simulink model "ASM_Traffic_MultiCore"  (R2026a)
settings: Solver=ode1  StartTime=SIM.tstart.v  StopTime=SIM.tend.v  FixedStep=SIM.StepSize.v
PostLoadFcn:
  | if any(exist('dsrtsu_mdlpostloadfcn', 'file') ~= 0), dsrtsu_mdlpostloadfcn('Execute', bdroot); end
  | try, asm_mdl_postloadfcn(bdroot, 'UpdateModel', 3600); catch, disp(lasterr); end,
InitFcn:
  | , if any(exist('rtifpga_mdlclblib', 'file') ~= 0), rtifpga_mdlclblib('Init', bdroot); end,
  | , if any(exist('dsmpb_private', 'file') ~= 0), dsmpb_private('dsmpb_mdlclblib', 'Init', bdroot); end,
model workspace (MAT data in the model file):
  asmReferencePath = [0 0.01 0.02 0.03 0.04 0.05 0.06 0.07 0.08 0.09 0.1 0.11 ... (350007 elements, 50001x7)]
  roadBounds : Simulink.Parameter (value not decoded)
  safetyAxes : Simulink.Parameter (value not decoded)
undefined symbols (not defined in the file): _to_, a0b2, ASM_BrakeHydraulics_DemoSystems, ASM_VehicleDynamics_DemoSystems, b98103fe8ad365046cd0, BrakeCircuit, controllerConfig, CPT, Crankshaft, DiscIntNeverNeededParam, dsmsi, FinalDriveAssembly, MDL, ModeSignals, mu, Pos_BrakePedal_Maneuver, rad, RefSignals, roadFamilyData, roadFamilyId, s_to_rpm, SIM, SoftECU, Suspension, Tire, Transmission
libraries: ASM_Traffic_lib x135, simulink x98, ASM_Utils_lib x77, ASM_VehicleDynamics_lib x70, ASM_Environment_lib x22, dsmpblib x20, dsmsilib x15, MDLD_Utils_lib x10, ASM_BrakeHydraulics_lib x3, sl_discontinuities x2
(part 4 of 65)

== system ASM_Traffic_MultiCore/ElectricalSystem/SignalInterface ==
  In : Inport
  ASMSignalInterface : Subsystem  mask(ASM_SIGNAL_INTERFACE){LabelTextfield=ElectricalSystem}
      mask prompts: LabelTextfield "Label"
      mask help:
      | The ASMSignalInterface block processes the ASMSignalBus and provides a vector-based interface for each signal (e.g. ModelDesk Plotting).
      |
      | Always push the update button after you have changed the signal bus structure in order to synchronize the signal interface. The update may take a few seconds.
      | A modified model must be reloaded in ModelDesk to keep consistency of ModelDesk and simulation model plot signals. Therefore select ''Update Model'' from the ''Simulation Model'' context menu of the ModelDesk Project Navigator.
      settings: AttributesFormatString=Label: %<LabelTextfield>
      settings: CopyFcn=|
      | try
      |  set_param(gcb,'LinkStatus', 'none')
      | catch
      | end
      mask Help: eval(['asm_modelhelp(gcbh,''tool'',''ASM_Utils_lib'', ''ASMSIGNALINTERFACE'')'])
      mask DialogControl Hint Prompt: For changes of Label first apply change and then push "Update".
      mask DialogControl UpdateButton Prompt: Update
      mask DialogControl UpdateButton Callback: asm_mdld_plot_block_update(bdroot(gcb), 'update', 'current');
      mask DialogControl UpdateAllButton Prompt: Update All
      mask DialogControl UpdateAllButton Callback: asm_mdld_plot_block_update(bdroot(gcb), 'update', 'all');
  Bus Selector Disable Signals : BusSelector  OutputSignals=ExternalModel.Sw_ModelDeskPlottingInterface[0Disabled|1Enabled]
  wires:
  Bus Selector Disable Signals/1 -> ASMSignalInterface/Enable  "<Sw_ModelDeskPlottingInterface[0Disabled|1Enabled]>"
  In/1 -> Bus Selector Disable Signals/1
  [ASMBUS_ElectricalSystem_Plant] -> ASMSignalInterface/1(ASMSignalBus)

== system ASM_Traffic_MultiCore/Engine/Control ==
  note: Engine Basic Control
  Interface_In : Inport
  Plant : Inport  Port=2
  SoftECU_Engine : Subsystem
  UserInterface : Subsystem
  Control : Outport  VectorParamsAs1DForOutWhenUnconnected=off
  wires:
  SoftECU_Engine/1(ASMSignalBus) -> UserInterface/1(In)
  UserInterface/1(Out) -> SoftECU_Engine/1(UserInterface)
  Plant/1 -> SoftECU_Engine/3(Plant)
  SoftECU_Engine/2(Out) -> Control/1
  Interface_In/1 -> SoftECU_Engine/2(Interface_In)

== system ASM_Traffic_MultiCore/Engine/Interface_In ==
  note: Engine Basic
  In : Inport
  Bus Creator : BusCreator  Inputs=1
  Bus Selector2 : BusSelector  OutputSignals=Environment.Plant.Sw_ModelPortBlocks[0Disabled|1Enabled],Environment.Plant.Sw_ModelDeskPlottingInterface[0Disabled|1Enabled],DomainControl.TorqueManager.Control.Ignition_ICE[0Off|1On],DomainControl.TorqueManager.Control.StarterReq_ICE[0Off|1On],Drivetrain.Control.Factor_Trq_Engine_Red[%],VehicleDynamics.Control.Enable_TrqDecrease_Fast_ESP[0|1],VehicleDynamics.Control.Trq_DecreaseRequest_Fast_ESP[Nm],VehicleDynamics.Control.Enable_TrqIncrease_ESP[0|1],VehicleDynamics.Control.Trq_IncreaseRequest_ESP[Nm],VehicleDynamics.Control.Enable_TrqDecrease_Slow_ESP[0|1],VehicleDynamics.Control.Trq_DecreaseRequest_Slow_ESP[Nm],DomainControl.TorqueManager.Control.Trq_Request_ICE[Nm],Driver.Plant.Pos_AccPedal[%],Environment.Plant.Reset_States[0|1],Drivetrain.Plant.n_Engine[rpm],Environment.Plant.State_StartButton[-1PowerOff|0Acc|1PowerOn|2StarterOn],DomainControl.TorqueManager.Control.Vehicle_Topology[-2|-1|0|2],VehicleDynamics.Plant.v_x_Vehicle_CoG[km|h],Drivetrain.Plant.Sw_CrankShaft_Reset[0Disabled|1Enabled],Environment.Plant.Mode_StartButtonState[1Stim|2SoftECU],DomainControl.DriverAssistance.Control.Enable_Trq_Increase_ACC[0|1],DomainControl.DriverAssistance.Control.Trq_IncreaseRequest_ACC[Nm]
  Enable_n_Engine_Idle_Request[0|1] : Constant  Value=0
  ModelSignals : Subsystem
  n_Engine_Idle_Request[rpm] : Constant  Value=0
  Out : Outport  VectorParamsAs1DForOutWhenUnconnected=off
  wires:
  Bus Selector2/2 -> ModelSignals/2(Sw_ModelDeskPlottingInterface[0Disabled|1Enabled])  "<Sw_ModelDeskPlottingInterface[0Disabled|1Enabled]>"
  Bus Selector2/1 -> ModelSignals/1(Sw_ModelPortBlocks[0Disabled|1Enabled])  "<Sw_ModelPortBlocks[0Disabled|1Enabled]>"
  In/1 -> Bus Selector2/1
  Bus Selector2/12 -> ModelSignals/12(Trq_Request_ICE[Nm])  "<Trq_Request_ICE[Nm]>"
  Bus Selector2/22 -> ModelSignals/22(Trq_Request_Extern2[Nm])  "<Trq_IncreaseRequest_ACC[Nm]>"
  Bus Selector2/21 -> ModelSignals/21(Enable_Trq_Request_Extern2[0|1])  "<Enable_Trq_Increase_ACC[0|1]>"
  Bus Selector2/7 -> ModelSignals/7(Trq_Decrease_Request_Fast_ESP[Nm])  "<Trq_DecreaseRequest_Fast_ESP[Nm]>"
  Bus Selector2/6 -> ModelSignals/6(Enable_Trq_Decrease_Fast_ESP[0|1])  "<Enable_TrqDecrease_Fast_ESP[0|1]>"
  Bus Selector2/5 -> ModelSignals/5(Factor_Trq_Engine_Red[%])  "<Factor_Trq_Engine_Red[%]>"
  Bus Selector2/4 -> ModelSignals/4(Sw_StarterReq[0Off|1On])  "<StarterReq_ICE[0Off|1On]>"
  Bus Selector2/3 -> ModelSignals/3(Sw_Ignition[0Off|1On])  "<Ignition_ICE[0Off|1On]>"
  Bus Selector2/11 -> ModelSignals/11(Trq_Request_Extern1[Nm])  "<Trq_DecreaseRequest_Slow_ESP[Nm]>"
  Bus Selector2/10 -> ModelSignals/10(Enable_Trq_Request_Extern1[0|1])  "<Enable_TrqDecrease_Slow_ESP[0|1]>"
  Bus Selector2/9 -> ModelSignals/9(Trq_Increase_Request_Fast_ESP[Nm])  "<Trq_IncreaseRequest_ESP[Nm]>"
  Bus Selector2/8 -> ModelSignals/8(Enable_Trq_Increase_Fast_ESP[0|1])  "<Enable_TrqIncrease_ESP[0|1]>"
  Bus Creator/1 -> Out/1
  Enable_n_Engine_Idle_Request[0|1]/1 -> ModelSignals/23(Enable_n_Engine_Idle_Request[0|1])
  n_Engine_Idle_Request[rpm]/1 -> ModelSignals/24(n_Engine_Idle_Request[rpm])
  Bus Selector2/13 -> ModelSignals/13(Pos_AccPedal_Driver[%])  "<Pos_AccPedal[%]>"
  Bus Selector2/14 -> ModelSignals/14(Reset_States[0|1])  "<Reset_States[0|1]>"
  Bus Selector2/15 -> ModelSignals/15(n_Engine[rpm])  "<n_Engine[rpm]>"
  Bus Selector2/16 -> ModelSignals/16(State_StartButton[-1|0|1|2])  "<State_StartButton[-1PowerOff|0Acc|1PowerOn|2StarterOn]>"
  Bus Selector2/17 -> ModelSignals/17(Vehicle_Topology[-2|-1|0|2])  "<Vehicle_Topology[-2|-1|0|2]>"
  Bus Selector2/18 -> ModelSignals/18(v_x_Vehicle[km|h])  "<v_x_Vehicle_CoG[km|h]>"
  Bus Selector2/19 -> ModelSignals/19(Sw_CrankShaft_Reset[0Disabled|1Enabled])  "<Sw_CrankShaft_Reset[0Disabled|1Enabled]>"
  Bus Selector2/20 -> ModelSignals/20(Mode_StartButtonState[1Stim|2SoftECU])  "<Mode_StartButtonState[1Stim|2SoftECU]>"
  ModelSignals/1(Out) -> Bus Creator/1

== system ASM_Traffic_MultiCore/Engine/Interface_Out ==
  note: Engine Basic
  In : Inport
  Bus Creator2 : BusCreator  Inputs=2
  Bus Selector2 : BusSelector  OutputSignals=Plant.Engine.Trq_Eff_Engine[Nm],Plant.Engine.Trq_Fric_Engine[Nm]
  Bus Selector6 : BusSelector  OutputSignals=Control.State_Engine[0|1|2|3|4],Control.n_Engine_Idle_Set[rpm],Control.Sw_Starter[0Off|1On],Control.Enable_Trq_Shift_Request[0|1],Control.Trq_Shift_Request[Nm]
  Control_ModelSignals : Subsystem
  CrankAngle_Cyl[aTDC] : Constant  Value=0
  EngOP_Num[] : Constant  Value=0
  Plant_ModelSignals : Subsystem
  Pos_AccPedal_Meas[%] : Constant  Value=0
  State_StartStop[1Off|2NotReady|3Ready|4EngStopped] : Constant
  Sw_Replace_Env[0|1] : Constant  Value=0
  T_Ambient[degC] : Constant  Value=23
  T_Coolant_ICE[degC] : Constant  Value=85
  Trq_MeanEff_Engine_Meas[Nm] : Constant  Value=0
  Type_Engine[0Unkown|1Other|2Otto|3Diesel|4Electric] : Constant
  n_Engine_Meas[rpm] : Constant  Value=0
  p_Ambient[Pa] : Constant  Value=1e5
  Out : Outport  VectorParamsAs1DForOutWhenUnconnected=off
  wires:
  CrankAngle_Cyl[aTDC]/1 -> Control_ModelSignals/7(CrankAngle_Cyl[aTDC])
  T_Ambient[degC]/1 -> Control_ModelSignals/9(T_Ambient[degC])
  p_Ambient[Pa]/1 -> Control_ModelSignals/8(p_Ambient[Pa])
  Trq_MeanEff_Engine_Meas[Nm]/1 -> Control_ModelSignals/14(Trq_MeanEff_Engine_Meas[Nm])
  n_Engine_Meas[rpm]/1 -> Control_ModelSignals/13(n_Engine_Meas[rpm])
  Pos_AccPedal_Meas[%]/1 -> Control_ModelSignals/12(Pos_AccPedal_Meas[%])
  EngOP_Num[]/1 -> Control_ModelSignals/11(EngOP_Num[])
  Sw_Replace_Env[0|1]/1 -> Control_ModelSignals/10(Sw_Replace_Env[0|1])
  Bus Selector6/2 -> Control_ModelSignals/2(n_Engine_Idle_Set[rpm])  "<n_Engine_Idle_Set[rpm]>"
  Bus Selector6/1 -> Control_ModelSignals/1(State_ICEngine[0|1|2|3|4])  "<State_Engine[0|1|2|3|4]>"
  State_StartStop[1Off|2NotReady|3Ready|4EngStopped]/1 -> Control_ModelSignals/6(State_StartStop[1Off|2NotReady|3Ready|4EngStopped])
  T_Coolant_ICE[degC]/1 -> Plant_ModelSignals/3(T_Coolant_ICE[degC])
  Bus Selector2/2 -> Plant_ModelSignals/2(Trq_Fric_Engine[Nm])  "<Trq_Fric_Engine[Nm]>"
  In/1 -> Bus Selector6/1, Bus Selector2/1
  Bus Selector2/1 -> Plant_ModelSignals/1(Trq_MeanEff_Engine[Nm])  "<Trq_Eff_Engine[Nm]>"
  Bus Creator2/1 -> Out/1  "Engine"
  Bus Selector6/3 -> Control_ModelSignals/3(Sw_Starter[0Off|1On])  "<Sw_Starter[0Off|1On]>"
  Bus Selector6/4 -> Control_ModelSignals/4(Enable_Trq_Shift_Request[0|1])  "<Enable_Trq_Shift_Request[0|1]>"
  Bus Selector6/5 -> Control_ModelSignals/5(Trq_Shift_Request[Nm])  "<Trq_Shift_Request[Nm]>"
  Control_ModelSignals/1(Out) -> Bus Creator2/1
  Plant_ModelSignals/1(Out) -> Bus Creator2/2
  Type_Engine[0Unkown|1Other|2Otto|3Diesel|4Electric]/1 -> Plant_ModelSignals/4(Type_Engine[0Unkown|1Other|2Otto|3Diesel|4Electric])

== system ASM_Traffic_MultiCore/Engine/Plant ==
  note: Engine Basic
  Interface_In : Inport
  Control : Inport  Port=2
  EngineBasic : Subsystem
  UserInterface : Subsystem
  Plant : Outport  VectorParamsAs1DForOutWhenUnconnected=off
  wires:
  Control/1 -> EngineBasic/3(Control)
  UserInterface/1(Out) -> EngineBasic/1(UserInterface)
  Interface_In/1 -> UserInterface/2(Interface_In), EngineBasic/2(Interface_In)
  EngineBasic/1(ASMSignalBus) -> Plant/1, UserInterface/1(In)

== system ASM_Traffic_MultiCore/Engine/SignalInterface ==
  In : Inport
  ASMSignalInterface : Subsystem  mask(ASM_SIGNAL_INTERFACE){LabelTextfield=Engine}
      mask prompts: LabelTextfield "Label"
      mask help:
      | The ASMSignalInterface block processes the ASMSignalBus and provides a vector-based interface for each signal (e.g. ModelDesk Plotting).
      |
      | Always push the update button after you have changed the signal bus structure in order to synchronize the signal interface. The update may take a few seconds.
      | A modified model must be reloaded in ModelDesk to keep consistency of ModelDesk and simulation model plot signals. Therefore select ''Update Model'' from the ''Simulation Model'' context menu of the ModelDesk Project Navigator.
      settings: AttributesFormatString=Label: %<LabelTextfield>
      settings: CopyFcn=|
      | try
      |  set_param(gcb,'LinkStatus', 'none')
      | catch
      | end
      mask Help: eval(['asm_modelhelp(gcbh,''tool'',''ASM_Utils_lib'', ''ASMSIGNALINTERFACE'')'])
      mask DialogControl Hint Prompt: For changes of Label first apply change and then push "Update".
      mask DialogControl UpdateButton Prompt: Update
      mask DialogControl UpdateButton Callback: asm_mdld_plot_block_update(bdroot(gcb), 'update', 'current');
      mask DialogControl UpdateAllButton Prompt: Update All
      mask DialogControl UpdateAllButton Callback: asm_mdld_plot_block_update(bdroot(gcb), 'update', 'all');
  Bus Creator : BusCreator  Inputs=2
  Bus Selector Disable Signals : BusSelector  OutputSignals=ExternalModel.Sw_ModelPortBlocks[0Disabled|1Enabled],ExternalModel.Sw_ModelDeskPlottingInterface[0Disabled|1Enabled]
  ExternalOutports : Subsystem  TreatAsAtomicUnit=on
  wires:
  Bus Selector Disable Signals/2 -> ASMSignalInterface/Enable  "<Sw_ModelDeskPlottingInterface[0Disabled|1Enabled]>"
  Bus Selector Disable Signals/1 -> ExternalOutports/Enable  "<Sw_ModelPortBlocks[0Disabled|1Enabled]>"
  In/1 -> Bus Selector Disable Signals/1
  Bus Creator/1 -> ASMSignalInterface/1(ASMSignalBus), ExternalOutports/1(In1)
  [ASMBUS_Engine_Control] -> Bus Creator/1
  [ASMBUS_Engine_Plant] -> Bus Creator/2

== system ASM_Traffic_MultiCore/Environment/GroundTruth ==
  note: GroundTruth
  In : Inport
  Bus Creator2 : BusCreator  Inputs=1
  PlantModel : Subsystem
  UserInterface : Subsystem
  Out : Outport  VectorParamsAs1DForOutWhenUnconnected=off
  wires:
  UserInterface/1(Out) -> PlantModel/1(UserInterface)
  In/1 -> PlantModel/2(In), UserInterface/1(Interface_In)
  PlantModel/1(ASMSignalBus) -> UserInterface/2(In), Bus Creator2/1
  Bus Creator2/1 -> Out/1  "GroundTruth"

== system ASM_Traffic_MultiCore/Environment/Interface_In ==
  note: Environment Traffic
  In : Inport
  Bus Creator1 : BusCreator  Inputs=1
  Bus Selector1 : BusSelector  OutputSignals=Environment.Plant.Sw_ModelPortBlocks[0Disabled|1Enabled],Environment.Plant.Sw_ModelDeskPlottingInterface[0Disabled|1Enabled],VehicleDynamics.Plant.Angle_SteeringWheel[deg],VehicleDynamics.Plant.Angle_SteeringWheel_dt[deg|s],VehicleDynamics.Plant.Trq_SteeringWheel[Nm],VehicleDynamics.Plant.r_Dyn_Tire[FL;FR;RL;RR][m],VehicleDynamics.Plant.Coef_RollingRes[FL;FR;RL;RR][],VehicleDynamics.Plant.CorneringStiffness[FL;FR;RL;RR][N],VehicleDynamics.Plant.Pos_Vehicle_CoorSys_E[x;y;z][m],VehicleDynamics.Plant.Angle_Vehicle_CoorSys_E[x;y;z][deg],VehicleDynamics.Plant.s_Vehicle[m],VehicleDynamics.Plant.v_x_Vehicle_CoG[km|h],VehicleDynamics.Plant.v_y_Vehicle_CoG[km|h],VehicleDynamics.Plant.RollRate_Vehicle_CoG[deg|s],VehicleDynamics.Plant.YawRate_Vehicle_CoG[deg|s],VehicleDynamics.Plant.a_y_Vehicle_CoG[m|s2],VehicleDynamics.Plant.RotationMatrix_V_to_E[1x9],VehicleDynamics.Plant.Const_r_unloaded_Tire_Mean[m],VehicleDynamics.Plant.Coef_RollingRes_Mean[],DomainControl.DriverAssistance.Control.AEB[0|1],DomainControl.DriverAssistance.Control.FCW[0|1],Driver.Plant.Pos_AccPedal[%],Driver.Plant.Pos_BrakePedal[%],Driver.Plant.Pos_ClutchPedal[%],Drivetrain.Plant.Gear[],Driver.Plant.SelectorLever[-3T|-2P|-1R|0N|1D],Driver.Plant.s_Preview[m],Driver.Plant.Angle_SteeringWheel[deg],Driver.Plant.t_Preview_vRef_Driver[s],Drivetrain.Plant.Type_Engine_1[0Unkown|1Other|2Otto|3Diesel|4Electric],Drivetrain.Plant.Trq_Engine_1[Nm],Drivetrain.Plant.n_Engine_1[rpm],Drivetrain.Plant.Type_Engine_2[0Unkown|1Other|2Otto|3Diesel|4Electric],Drivetrain.Plant.Trq_Engine_2[Nm],Drivetrain.Plant.n_Engine_2[rpm],VehicleDynamics.Plant.m_TotalVehicle[kg],DomainControl.StartSystem.Control.State_StartButton[-2|-1|0|1|2|3],DomainControl.DriverAssistance.Control.ACC_State[1OFF|2Standby|3ON],DomainControl.DriverAssistance.Control.Driver_Override_ACC_Active[0Off|1On],DomainControl.DriverAssistance.Control.Driver_Override_ACC_Reason[0NoOverride|1BrakePedal|2AccPedal],VehicleDynamics.Plant.omega_Wheel[rad|s],VehicleDynamics.Plant.Slip_x_Wheel[],VehicleDynamics.Plant.Pos_CP_FL_CoorSys_E[x;y][m],VehicleDynamics.Plant.Pos_CP_FR_CoorSys_E[x;y][m],VehicleDynamics.Plant.Pos_CP_RL_CoorSys_E[x;y][m],VehicleDynamics.Plant.Pos_CP_RL2_CoorSys_E[x;y][m],VehicleDynamics.Plant.Pos_CP_RR_CoorSys_E[x;y][m],VehicleDynamics.Plant.Pos_CP_RR2_CoorSys_E[x;y][m],VehicleDynamics.Plant.Pos_CP_R2L_CoorSys_E[x;y][m],VehicleDynamics.Plant.Pos_CP_R2L2_CoorSys_E[x;y][m],VehicleDynamics.Plant.Pos_CP_R2R_CoorSys_E[x;y][m],VehicleDynamics.Plant.Pos_CP_R2R2_CoorSys_E[x;y][m],Drivetrain.Plant.Mode_Transmission[1Manual|2Automatic],Drivetrain.Plant.Mode_Drivetrain[1|2|3|4|5],VehicleDynamics.Plant.Sw_MasterBrakeCylinder_Mode[1linear|2physical|3Booster],VehicleDynamics.Plant.Active_CP_VehDyn[],VehicleDynamics.Plant.Pos_CP_Front_CoorSys_E[x;y][m],VehicleDynamics.Plant.Pos_CP_Rear_CoorSys_E[x;y][m]
  ModelSignals : Subsystem
  Pos_CP_FL2_Trailer_CoorSys_E[x;y][m] : Constant  Value=[0;0]
  Pos_CP_FL_Trailer_CoorSys_E[x;y][m] : Constant  Value=[0;0]
  Pos_CP_FR2_Trailer_CoorSys_E[x;y][m] : Constant  Value=[0;0]
  Pos_CP_FR_Trailer_CoorSys_E[x;y][m] : Constant  Value=[0;0]
  Pos_CP_R2L2_Trailer_CoorSys_E[x;y][m] : Constant  Value=[0;0]
  Pos_CP_R2L_Trailer_CoorSys_E[x;y][m] : Constant  Value=[0;0]
  Pos_CP_R2R2_Trailer_CoorSys_E[x;y][m] : Constant  Value=[0;0]
  Pos_CP_R2R_Trailer_CoorSys_E[x;y][m] : Constant  Value=[0;0]
  Pos_CP_RL2_Trailer_CoorSys_E[x;y][m] : Constant  Value=[0;0]
  Pos_CP_RL_Trailer_CoorSys_E[x;y][m] : Constant  Value=[0;0]
  Pos_CP_RR2_Trailer_CoorSys_E[x;y][m] : Constant  Value=[0;0]
  Pos_CP_RR_Trailer_CoorSys_E[x;y][m] : Constant  Value=[0;0]
  Out : Outport  VectorParamsAs1DForOutWhenUnconnected=off
  wires:
  Bus Creator1/1 -> Out/1  "Interface_In"
  ModelSignals/1(Out) -> Bus Creator1/1
  Pos_CP_FL_Trailer_CoorSys_E[x;y][m]/1 -> ModelSignals/57(Pos_CP_FL_Trailer_CoorSys_E[x;y][m])
  Pos_CP_FL2_Trailer_CoorSys_E[x;y][m]/1 -> ModelSignals/58(Pos_CP_FL2_Trailer_CoorSys_E[x;y][m])
  Pos_CP_FR_Trailer_CoorSys_E[x;y][m]/1 -> ModelSignals/59(Pos_CP_FR_Trailer_CoorSys_E[x;y][m])
  Pos_CP_FR2_Trailer_CoorSys_E[x;y][m]/1 -> ModelSignals/60(Pos_CP_FR2_Trailer_CoorSys_E[x;y][m])
  Pos_CP_RL_Trailer_CoorSys_E[x;y][m]/1 -> ModelSignals/61(Pos_CP_RL_Trailer_CoorSys_E[x;y][m])
  Pos_CP_RL2_Trailer_CoorSys_E[x;y][m]/1 -> ModelSignals/62(Pos_CP_RL2_Trailer_CoorSys_E[x;y][m])
  Pos_CP_RR_Trailer_CoorSys_E[x;y][m]/1 -> ModelSignals/63(Pos_CP_RR_Trailer_CoorSys_E[x;y][m])
  Pos_CP_RR2_Trailer_CoorSys_E[x;y][m]/1 -> ModelSignals/64(Pos_CP_RR2_Trailer_CoorSys_E[x;y][m])
  Pos_CP_R2L_Trailer_CoorSys_E[x;y][m]/1 -> ModelSignals/65(Pos_CP_R2L_Trailer_CoorSys_E[x;y][m])
  Pos_CP_R2L2_Trailer_CoorSys_E[x;y][m]/1 -> ModelSignals/66(Pos_CP_R2L2_Trailer_CoorSys_E[x;y][m])
  Pos_CP_R2R_Trailer_CoorSys_E[x;y][m]/1 -> ModelSignals/67(Pos_CP_R2R_Trailer_CoorSys_E[x;y][m])
  Pos_CP_R2R2_Trailer_CoorSys_E[x;y][m]/1 -> ModelSignals/68(Pos_CP_R2R2_Trailer_CoorSys_E[x;y][m])
  Bus Selector1/1 -> ModelSignals/1(Sw_ModelPortBlocks[0Disabled|1Enabled])  "<Sw_ModelPortBlocks[0Disabled|1Enabled]>"
  Bus Selector1/2 -> ModelSignals/2(Sw_ModelDeskPlottingInterface[0Disabled|1Enabled])  "<Sw_ModelDeskPlottingInterface[0Disabled|1Enabled]>"
  Bus Selector1/3 -> ModelSignals/3(Angle_SteeringWheel_SteeringSystem[deg])  "<Angle_SteeringWheel[deg]>"
  Bus Selector1/4 -> ModelSignals/4(Angle_SteeringWheel_dt_SteeringSystem[deg|s])  "<Angle_SteeringWheel_dt[deg|s]>"
  Bus Selector1/5 -> ModelSignals/5(Trq_SteeringWheel_SteeringSystem[Nm])  "<Trq_SteeringWheel[Nm]>"
  Bus Selector1/6 -> ModelSignals/6(r_Dyn_Tire[FL;FR;RL;RR][m])  "<r_Dyn_Tire[FL;FR;RL;RR][m]>"
  Bus Selector1/7 -> ModelSignals/7(Coef_RollingRes[FL;FR;RL;RR][])  "<Coef_RollingRes[FL;FR;RL;RR][]>"
  Bus Selector1/8 -> ModelSignals/8(CorneringStiffness[FL;FR;RL;RR][N])  "<CorneringStiffness[FL;FR;RL;RR][N]>"
  Bus Selector1/9 -> ModelSignals/9(Pos_Vehicle_CoorSys_E[x;y;z][m])  "<Pos_Vehicle_CoorSys_E[x;y;z][m]>"
  Bus Selector1/10 -> ModelSignals/10(Angle_Vehicle_CoorSys_E[x;y;z][deg])  "<Angle_Vehicle_CoorSys_E[x;y;z][deg]>"
  Bus Selector1/11 -> ModelSignals/11(s_Vehicle[m])  "<s_Vehicle[m]>"
  Bus Selector1/12 -> ModelSignals/12(v_x_Vehicle_CoG[km|h])  "<v_x_Vehicle_CoG[km|h]>"
  Bus Selector1/13 -> ModelSignals/13(v_y_Vehicle_CoG[km|h])  "<v_y_Vehicle_CoG[km|h]>"
  Bus Selector1/14 -> ModelSignals/14(RollRate_Vehicle_CoG[deg|s])  "<RollRate_Vehicle_CoG[deg|s]>"
  Bus Selector1/15 -> ModelSignals/15(YawRate_Vehicle_CoG[deg|s])  "<YawRate_Vehicle_CoG[deg|s]>"
  Bus Selector1/16 -> ModelSignals/16(a_y_Vehicle_CoG[m|s2])  "<a_y_Vehicle_CoG[m|s2]>"
  Bus Selector1/17 -> ModelSignals/17(RotationMatrix_V_to_E[1x9])  "<RotationMatrix_V_to_E[1x9]>"
  Bus Selector1/18 -> ModelSignals/18(Const_r_unloaded_Tire_Mean[m])  "<Const_r_unloaded_Tire_Mean[m]>"
  Bus Selector1/19 -> ModelSignals/19(Coef_RollingRes_Mean[])  "<Coef_RollingRes_Mean[]>"
  Bus Selector1/20 -> ModelSignals/20(AEB[0|1])  "<AEB[0|1]>"
  Bus Selector1/21 -> ModelSignals/21(FCW[0|1])  "<FCW[0|1]>"
  Bus Selector1/22 -> ModelSignals/22(Pos_AccPedal[%])  "<Pos_AccPedal[%]>"
  Bus Selector1/23 -> ModelSignals/23(Pos_BrakePedal[%])  "<Pos_BrakePedal[%]>"
  Bus Selector1/24 -> ModelSignals/24(Pos_ClutchPedal[%])  "<Pos_ClutchPedal[%]>"
  Bus Selector1/25 -> ModelSignals/25(Gear[])  "<Gear[]>"
  Bus Selector1/26 -> ModelSignals/26(SelectorLever[-3T|-2P|-1R|0N|1D])  "<SelectorLever[-3T|-2P|-1R|0N|1D]>"
  Bus Selector1/27 -> ModelSignals/27(s_Preview[m])  "<s_Preview[m]>"
  Bus Selector1/28 -> ModelSignals/28(Angle_SteeringWheel[deg])  "<Angle_SteeringWheel[deg]>"
  Bus Selector1/29 -> ModelSignals/29(t_Preview_vRef_Driver[s])  "<t_Preview_vRef_Driver[s]>"
  Bus Selector1/30 -> ModelSignals/30(Type_Engine_1[0Unkown|1Other|2Otto|3Diesel|4Electric])  "<Type_Engine_1[0Unkown|1Other|2Otto|3Diesel|4Electric]>"
  Bus Selector1/31 -> ModelSignals/31(Trq_Engine_1[Nm])  "<Trq_Engine_1[Nm]>"
  Bus Selector1/32 -> ModelSignals/32(n_Engine_1[rpm])  "<n_Engine_1[rpm]>"
  Bus Selector1/33 -> ModelSignals/33(Type_Engine_2[0Unkown|1Other|2Otto|3Diesel|4Electric])  "<Type_Engine_2[0Unkown|1Other|2Otto|3Diesel|4Electric]>"
  Bus Selector1/34 -> ModelSignals/34(Trq_Engine_2[Nm])  "<Trq_Engine_2[Nm]>"
  Bus Selector1/35 -> ModelSignals/35(n_Engine_2[rpm])  "<n_Engine_2[rpm]>"
  Bus Selector1/36 -> ModelSignals/36(m_TotalVehicle[kg])  "<m_TotalVehicle[kg]>"
  Bus Selector1/37 -> ModelSignals/37(State_StartButton[-2|-1|0|1|2|3])  "<State_StartButton[-2|-1|0|1|2|3]>"
  Bus Selector1/38 -> ModelSignals/38(ACC_State[1OFF|2Standby|3ON])  "<ACC_State[1OFF|2Standby|3ON]>"
  Bus Selector1/39 -> ModelSignals/39(Driver_Override_ACC_Active[0Off|1On])  "<Driver_Override_ACC_Active[0Off|1On]>"
  Bus Selector1/40 -> ModelSignals/40(Driver_Override_ACC_Reason[0NoOverride|1BrakePedal|2AccPedal])  "<Driver_Override_ACC_Reason[0NoOverride|1BrakePedal|2AccPedal]>"
  Bus Selector1/41 -> ModelSignals/41(omega_Wheel[rad|s])  "<omega_Wheel[rad|s]>"
  Bus Selector1/42 -> ModelSignals/42(Slip_x_Wheel[])  "<Slip_x_Wheel[]>"
  Bus Selector1/43 -> ModelSignals/43(Pos_CP_FL_CoorSys_E[x;y][m])  "<Pos_CP_FL_CoorSys_E[x;y][m]>"
  Bus Selector1/44 -> ModelSignals/44(Pos_CP_FR_CoorSys_E[x;y][m])  "<Pos_CP_FR_CoorSys_E[x;y][m]>"
  Bus Selector1/45 -> ModelSignals/45(Pos_CP_RL_CoorSys_E[x;y][m])  "<Pos_CP_RL_CoorSys_E[x;y][m]>"
  Bus Selector1/46 -> ModelSignals/46(Pos_CP_RL2_CoorSys_E[x;y][m])  "<Pos_CP_RL2_CoorSys_E[x;y][m]>"
  Bus Selector1/47 -> ModelSignals/47(Pos_CP_RR_CoorSys_E[x;y][m])  "<Pos_CP_RR_CoorSys_E[x;y][m]>"
  Bus Selector1/48 -> ModelSignals/48(Pos_CP_RR2_CoorSys_E[x;y][m])  "<Pos_CP_RR2_CoorSys_E[x;y][m]>"
  Bus Selector1/49 -> ModelSignals/49(Pos_CP_R2L_CoorSys_E[x;y][m])  "<Pos_CP_R2L_CoorSys_E[x;y][m]>"
  Bus Selector1/50 -> ModelSignals/50(Pos_CP_R2L2_CoorSys_E[x;y][m])  "<Pos_CP_R2L2_CoorSys_E[x;y][m]>"
  Bus Selector1/51 -> ModelSignals/51(Pos_CP_R2R_CoorSys_E[x;y][m])  "<Pos_CP_R2R_CoorSys_E[x;y][m]>"
  Bus Selector1/52 -> ModelSignals/52(Pos_CP_R2R2_CoorSys_E[x;y][m])  "<Pos_CP_R2R2_CoorSys_E[x;y][m]>"
  Bus Selector1/53 -> ModelSignals/53(Mode_Transmission[1Manual|2Automatic])  "<Mode_Transmission[1Manual|2Automatic]>"
  Bus Selector1/54 -> ModelSignals/54(Mode_Drivetrain[1|2|3|4|5])  "<Mode_Drivetrain[1|2|3|4|5]>"
  Bus Selector1/55 -> ModelSignals/55(Sw_MasterBrakeCylinder_Mode[1linear|2physical|3Booster])  "<Sw_MasterBrakeCylinder_Mode[1linear|2physical|3Booster]>"
  Bus Selector1/56 -> ModelSignals/56(Active_CP_VehDyn_Trailer[])  "<Active_CP_VehDyn[]>"
  Bus Selector1/57 -> ModelSignals/69(Pos_CP_Front_CoorSys_E[x;y][m])  "<Pos_CP_Front_CoorSys_E[x;y][m]>"
  Bus Selector1/58 -> ModelSignals/70(Pos_CP_Rear_CoorSys_E[x;y][m])  "<Pos_CP_Rear_CoorSys_E[x;y][m]>"
  In/1 -> Bus Selector1/1
